simulink model "servomotor"  (R2026b)
settings: Solver=VariableStepAuto  StopTime=5
model workspace (MAT data in the model file):
  b = 0.0005
  j = 5e-05
  k = 0.2
  ki = 7.33
  kp = 9.39
  l = 0.01
  r = 4
  ts = 0.01
  v = 7.4
libraries: SignalEditorBlockLib x1
settings Model: Creator=Amaan  LastModifiedBy=Amaan

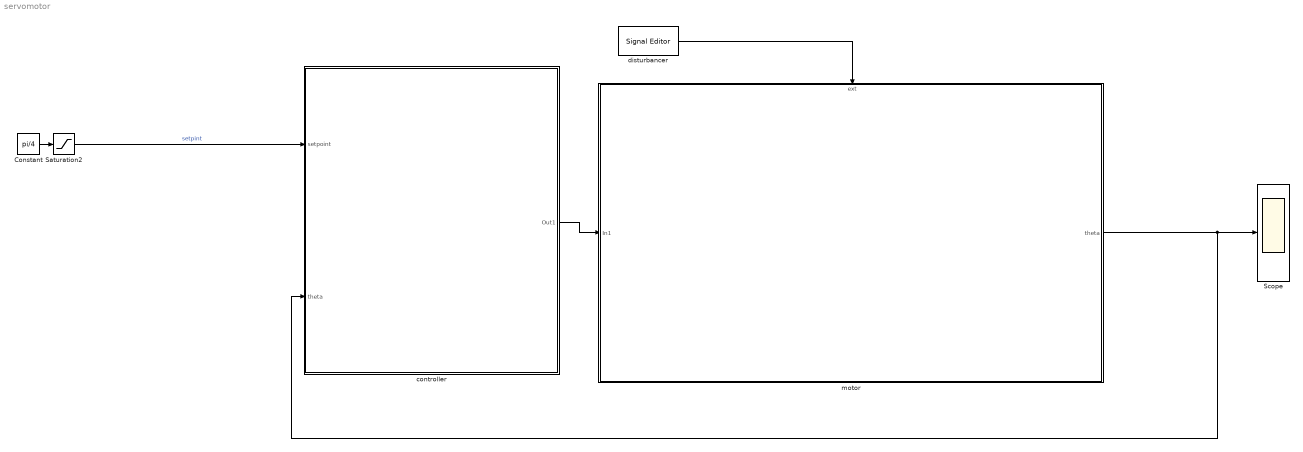
== system servomotor ==
  Constant : Constant  Value=pi/4
  Saturation2 : Saturate  UpperLimit=pi/4  LowerLimit=-pi/4
  Scope : Scope
      settings: ActiveDisplayYMinimum=-0.51358837887461073  ActiveDisplayYMaximum=1.3453665185987067
  controller : Subsystem  TreatAsAtomicUnit=on  mask{kp=9.39, ki=7.33, ts=0.01}
      mask prompts: kp "propotional gain"; ki "integral gain"; ts "sample time"
  disturbancer : SignalEditorBlockLib/Signal Editor  FileName=C:\Users\Amaan\Desktop\matlab\module 1\airleontesting.mat  ActiveScenario=calmAir  ActiveSignal=disturbance  IsBus=off  OutputBusObjectStr=Bus: BusObject  SampleTime=0  ZeroCross=off  OutputAfterFinalValue=Setting to zero  Unit=inherit  PreserveSignalName=on  ApplySigPropsToAllScenarios=off  ApplySigPropsToAllSignals=off  SignalPropertySource=Signal data in MAT file
  motor : Subsystem
      settings: PortSchema="{\"entries\":[{\"content\":{\"sides\":[{\"content\":{\"connectorIds\":[\"In1\"]},\"type\":\"ConnectorPlacement.EquallySpacedRectSide\",\"uuid\":\"a0fe10d6-0743-4278-bc56-fa92d978892d\"},{\"content\":{\"connectorIds\":[\"Out1\"],\"side\":\"RIGHT\"},\"type\":\"ConnectorPlacement.EquallySpacedRectSide\",\"uuid\":\"380184e0-b0b3-4ca5-a248-da8a50f56b9f\"},{\"content\":{\"connectorIds\":[\"In2\"],\"side\":\"TOP\"},\"type\":\"ConnectorPlacement.EquallySpacedRectSide\",\"uuid\":\"1f587022-4e17-425d-af03-f535c87a9e2b\"}]},\"type\":\"ConnectorPlacement.EquallySpacedConnector\",\"uuid\":\"86c4c905-85e4-4036-8df4-ab807e60f4b1\"}],\"packageUris\":[\"http://schema.mathworks.com/mf0/Connector/R2020b\"],\"version\":\"1.0\"}"
  wires:
  Constant/1 -> Saturation2/1
  motor/1(theta) -> Scope/1, controller/2(theta)
  Saturation2/1 -> controller/1(setpoint)  "setpint"
  controller/1(Out1) -> motor/1(In1)
  disturbancer/1 -> motor/2(ext)

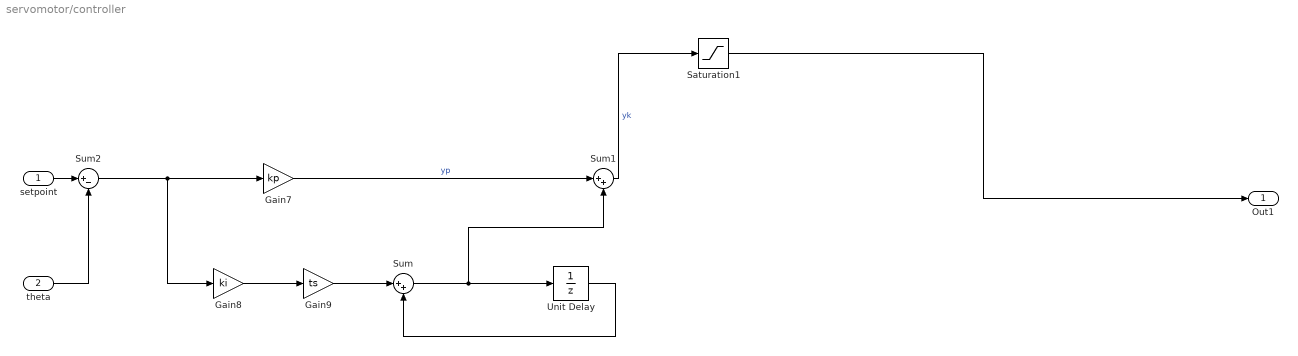
== system servomotor/controller ==
  setpoint : Inport
  theta : Inport  Port=2
  Gain7 : Gain  Gain=kp
  Gain8 : Gain  Gain=ki
  Gain9 : Gain  Gain=ts
  Saturation1 : Saturate  UpperLimit=v  LowerLimit=-v
  Sum : Sum  Inputs=|++
  Sum1 : Sum  Inputs=|++
  Sum2 : Sum  Inputs=|+-
  Unit Delay : UnitDelay  SampleTime=ts
  Out1 : Outport
  wires:
  Gain7/1 -> Sum1/1  "yp"
  Sum2/1 -> Gain8/1, Gain7/1
  Sum/1 -> Sum1/2, Unit Delay/1
  Unit Delay/1 -> Sum/2
  Gain8/1 -> Gain9/1
  Sum1/1 -> Saturation1/1  "yk"
  Saturation1/1 -> Out1/1
  Gain9/1 -> Sum/1
  setpoint/1 -> Sum2/1
  theta/1 -> Sum2/2

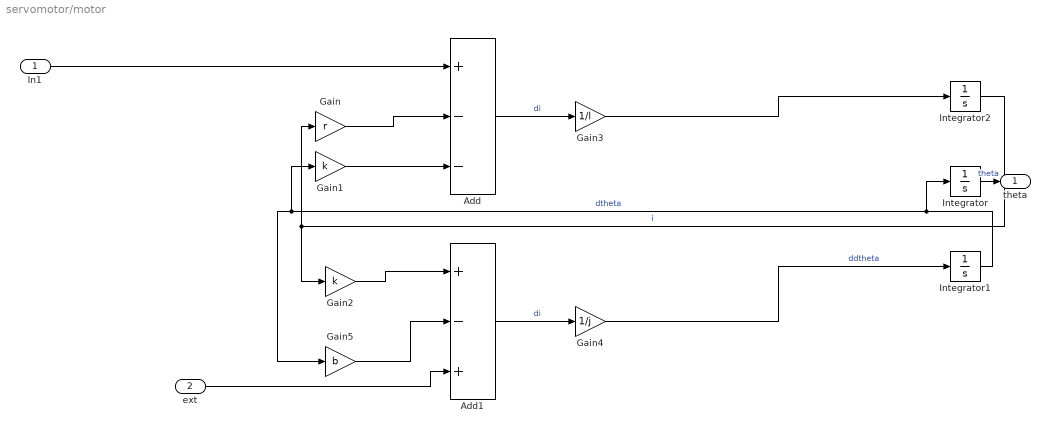
== system servomotor/motor ==
  In1 : Inport
  ext : Inport  Port=2
  Add : Sum  Inputs=+--
  Add1 : Sum  Inputs=+-+
  Gain : Gain  Gain=r
  Gain1 : Gain  Gain=k
  Gain2 : Gain  Gain=k
  Gain3 : Gain  Gain=1/l
  Gain4 : Gain  Gain=1/j
  Gain5 : Gain  Gain=b
  Integrator : Integrator
  Integrator1 : Integrator
  Integrator2 : Integrator
  theta : Outport
  wires:
  Integrator2/1 -> Gain/1, Gain2/1  "i"
  Add/1 -> Gain3/1  "di"
  Add1/1 -> Gain4/1  "di"
  Gain3/1 -> Integrator2/1
  In1/1 -> Add/1
  Integrator1/1 -> Gain1/1, Gain5/1, Integrator/1  "dtheta"
  Gain1/1 -> Add/3
  Gain2/1 -> Add1/1
  Gain/1 -> Add/2
  Gain4/1 -> Integrator1/1  "ddtheta"
  Gain5/1 -> Add1/2
  Integrator/1 -> theta/1  "theta"
  ext/1 -> Add1/3
